simulink library "Lib_Piccolo"  (R2018b)
settings: Solver=VariableStepAuto  StartTime=0.0  StopTime=10.0  RelTol=1e-3
values from neighbouring files (symbols this model uses):
  AccelErrInt2Brakes = 0.15    [SimulationControlConfig16P.m]    (also in SimulationControlConfig16P_LEGACY.m; SimulationControlConfigTAILLESS.m = 0.2; SimulationControlConfigUTAIL.m = 0.2)
  AileronMax = 25    [SimulationControlConfig16P.m]    (also in SimulationControlConfig16P_LEGACY.m; SimulationControlConfigTAILLESS.m; SimulationControlConfigUTAIL.m)
  AileronPower = 0.00268    [SimulationControlConfig16P.m]    (also in SimulationControlConfig16P_LEGACY.m; SimulationControlConfigTAILLESS.m; SimulationControlConfigUTAIL.m)
  AileronSurfaceMax = 45    [SimulationControlConfig16P.m]    (also in SimulationControlConfig16P_LEGACY.m)
  AileronTrim = 0    [SimulationControlConfig16P.m]    (also in SimulationControlConfig16P_LEGACY.m; SimulationControlConfigTAILLESS.m; SimulationControlConfigUTAIL.m)
  Alt = 1000 + TerrainHeight    [SimulationStateConfig.m]
  AltCruise_m = testPlans(testIndx).terrainElevation * 0.3048 + 200    [SimulationControlConfig16P.m]    (also in SimulationControlConfigTAILLESS.m = 1083; SimulationControlConfigUTAIL.m = testPlans(testIndx).terrainElevation * 0.3048 + 152)
  AltitudeRate2PitchCmdIntegratorInit = 0.1    [SimulationControlPre.m]
  AltMax = 10000    [SimulationControlConfig16P.m]    (also in SimulationControlConfig16P_LEGACY.m; SimulationControlConfigTAILLESS.m; SimulationControlConfigUTAIL.m)
  AltMaxAccel = 1.25    [SimulationControlConfig16P.m]    (also in SimulationControlConfig16P_LEGACY.m = 0.9; SimulationControlConfigTAILLESS.m = 1.7; SimulationControlConfigUTAIL.m = 2)
  AltMin = 0    [SimulationControlConfig16P.m]    (also in SimulationControlConfig16P_LEGACY.m; SimulationControlConfigTAILLESS.m; SimulationControlConfigUTAIL.m)
  AltRateCmd2Pitch = 0.50    (= 0.5)    [SimulationControlConfig16P.m]    (also in SimulationControlConfig16P_LEGACY.m = 0.6; SimulationControlConfigTAILLESS.m = 0.2; SimulationControlConfigUTAIL.m = 0.3)
  AltRateError2Pitch = 0.40    (= 0.4)    [SimulationControlConfig16P.m]    (also in SimulationControlConfig16P_LEGACY.m; SimulationControlConfigTAILLESS.m = 0.55; SimulationControlConfigUTAIL.m = 0.55)
  AltRateErrorInt2Pitch = 0.50    (= 0.5)    [SimulationControlConfig16P.m]    (also in SimulationControlConfig16P_LEGACY.m = 0.45; SimulationControlConfigTAILLESS.m; SimulationControlConfigUTAIL.m = 0.75)
  AltRateLpfCutOff = 3    [SimulationControlConfig16P.m]    (also in SimulationControlConfig16P_LEGACY.m; SimulationControlConfigTAILLESS.m = 2; SimulationControlConfigUTAIL.m = 2)
  AutoNosegear2Rudder = 26    [SimulationControlConfig16P.m]    (also in SimulationControlConfig16P_LEGACY.m; SimulationControlConfigTAILLESS.m = 25.2; SimulationControlConfigUTAIL.m = 14)
  b = 5.54    [SimulationControlConfig16P.m]    (also in SimulationControlConfig16P_LEGACY.m; SimulationControlConfigTAILLESS.m = 2.37; SimulationControlConfigUTAIL.m = 2.37)
  Bank2AileronIntegratorInit = 0    [SimulationControlPre.m]
  BankMax_User = BankMax_User/180*pi    (= 0.523598775598)    [SimulationControlConfig16P.m]    (also in SimulationControlConfig16P_LEGACY.m; SimulationControlConfigTAILLESS.m = 0.610865238198; SimulationControlConfigUTAIL.m = 0.628318530718)
  baseLegFlaps = 20    [SimulationControlConfig16P.m]    (also in SimulationControlConfig16P_LEGACY.m = 0; SimulationControlConfigTAILLESS.m = 15; SimulationControlConfigUTAIL.m = 10)
  C = GeneticOpt.C    [SimulationCostFunction.m]
  c = Sw/b    (= 0.841696750903)    [SimulationControlConfig16P.m]    (also in SimulationControlConfig16P_LEGACY.m; SimulationControlConfigTAILLESS.m = 0.354008438819; SimulationControlConfigUTAIL.m = 0.354008438819)
  cell2WheelFactorMG = 5.98    [SimulationSensorConfig16P_LEGACY.m]
  cell2WheelFactorNG = 1    [SimulationSensorConfig16P_LEGACY.m]
  cellSatMaxMG = 15000    [SimulationSensorConfig16P.m]    (also in SimulationSensorConfig16P_LEGACY.m; SimulationSensorConfigTAILLESS7P.m; SimulationSensorConfigUTAIL7P.m)
  cellSatMaxNG = 1000    [SimulationSensorConfig16P.m]    (also in SimulationSensorConfig16P_LEGACY.m; SimulationSensorConfigTAILLESS7P.m; SimulationSensorConfigUTAIL7P.m)
  cellSatMinMG = -15000    [SimulationSensorConfig16P.m]    (also in SimulationSensorConfig16P_LEGACY.m; SimulationSensorConfigTAILLESS7P.m; SimulationSensorConfigUTAIL7P.m)
  cellSatMinNG = -1000    [SimulationSensorConfig16P.m]    (also in SimulationSensorConfig16P_LEGACY.m; SimulationSensorConfigTAILLESS7P.m; SimulationSensorConfigUTAIL7P.m)
  CL_Limit = CL_Max    (= 0.54)    [SimulationControlConfig16P.m]    (also in SimulationControlConfig16P_LEGACY.m; SimulationControlConfigTAILLESS.m; SimulationControlConfigUTAIL.m = 0.53)
  CL_Max = 0.54    [SimulationControlConfig16P.m]    (also in SimulationControlConfig16P_LEGACY.m; SimulationControlConfigTAILLESS.m; SimulationControlConfigUTAIL.m = 0.53)
  CL_Max_Nom = 0.465    [SimulationControlConfig16P.m]    (also in SimulationControlConfig16P_LEGACY.m; SimulationControlConfigTAILLESS.m = 0.39; SimulationControlConfigUTAIL.m)
  CL_Min = 0    [SimulationControlConfig16P.m]    (also in SimulationControlConfig16P_LEGACY.m; SimulationControlConfigTAILLESS.m; SimulationControlConfigUTAIL.m)
  ClimbMaxFraction = 0.35    [SimulationControlConfig16P.m]    (also in SimulationControlConfig16P_LEGACY.m = 0.24; SimulationControlConfigTAILLESS.m = 0.19; SimulationControlConfigUTAIL.m = 0.21)
  ClimboutMaxBank = 7.0    (= 7)    [SimulationControlConfig16P.m]    (also in SimulationControlConfig16P_LEGACY.m; SimulationControlConfigTAILLESS.m = 5; SimulationControlConfigUTAIL.m)
  ClimboutTimer = 7.0    (= 7)    [SimulationControlConfig16P.m]    (also in SimulationControlConfig16P_LEGACY.m; SimulationControlConfigTAILLESS.m; SimulationControlConfigUTAIL.m)
  dCl_per_dFlap = 0.005581818    [SimulationControlConfig16P.m]    (also in SimulationControlConfig16P_LEGACY.m = 0; SimulationControlConfigTAILLESS.m = 0; SimulationControlConfigUTAIL.m = 0)
  DecelerationCmd = 3.1    [SimulationControlConfig16P.m]    (also in SimulationControlConfig16P_LEGACY.m; SimulationControlConfigTAILLESS.m = 0.1; SimulationControlConfigUTAIL.m = 0.1)
  DeRotateLogicEndTimer = abs((NoseDownLimit_Deg-1)/DeRotateRamp_Dps)    [SimulationControlConfig16P.m]    (also in SimulationControlConfig16P_LEGACY.m; SimulationControlConfigTAILLESS.m; SimulationControlConfigUTAIL.m)
  DeRotateLogicHoldNoseUpTimer = 0.1    [SimulationControlConfig16P.m]    (also in SimulationControlConfig16P_LEGACY.m; SimulationControlConfigTAILLESS.m; SimulationControlConfigUTAIL.m)
  DeRotateLogicTimerTimeout = 2    [SimulationControlConfig16P.m]    (also in SimulationControlConfig16P_LEGACY.m; SimulationControlConfigTAILLESS.m; SimulationControlConfigUTAIL.m)
  DeRotateLowerCmdSaturation = 0    [SimulationControlConfig16P.m]    (also in SimulationControlConfig16P_LEGACY.m; SimulationControlConfigTAILLESS.m; SimulationControlConfigUTAIL.m)
  DeRotateRamp_Dps = 3    [SimulationControlConfig16P.m]    (also in SimulationControlConfig16P_LEGACY.m; SimulationControlConfigTAILLESS.m = 8; SimulationControlConfigUTAIL.m = 8)
  DeRotateUpperCmdSaturation = 7    [SimulationControlConfig16P.m]    (also in SimulationControlConfig16P_LEGACY.m; SimulationControlConfigTAILLESS.m; SimulationControlConfigUTAIL.m)
  DescentMaxFraction = 0.22    [SimulationControlConfig16P.m]    (also in SimulationControlConfig16P_LEGACY.m = 0.2; SimulationControlConfigTAILLESS.m = 0.17; SimulationControlConfigUTAIL.m = 0.17)
  DesktopSimTerrainOffset_m = 0.406    [SimulationAircraftConfig.m]
  downwindFlaps = 0    [SimulationControlConfig16P.m]    (also in SimulationControlConfig16P_LEGACY.m; SimulationControlConfigTAILLESS.m; SimulationControlConfigUTAIL.m)
  DP_init = 0.5*1.225*V_init^2    [SimulationControlConfig16P.m]    (also in SimulationControlConfig16P_LEGACY.m; SimulationControlConfigTAILLESS.m; SimulationControlConfigUTAIL.m)
  dscNoiseMG = 1    [SimulationSensorConfig16P_LEGACY.m]
  dscNoiseNG = 0.25    [SimulationSensorConfig16P_LEGACY.m]
  DSCnumBits = 24    [SimulationSensorConfig16P.m]    (also in SimulationSensorConfig16P_LEGACY.m; SimulationSensorConfigTAILLESS7P.m; SimulationSensorConfigUTAIL7P.m)
  DSCRangeMaxMG = 15000    [SimulationSensorConfig16P.m]    (also in SimulationSensorConfig16P_LEGACY.m; SimulationSensorConfigTAILLESS7P.m; SimulationSensorConfigUTAIL7P.m)
  DSCRangeMaxNG = 1000    [SimulationSensorConfig16P.m]    (also in SimulationSensorConfig16P_LEGACY.m; SimulationSensorConfigTAILLESS7P.m; SimulationSensorConfigUTAIL7P.m)
  DSCRangeMinMG = -15000    [SimulationSensorConfig16P.m]    (also in SimulationSensorConfig16P_LEGACY.m; SimulationSensorConfigTAILLESS7P.m; SimulationSensorConfigUTAIL7P.m)
  DSCRangeMinNG = -1000    [SimulationSensorConfig16P.m]    (also in SimulationSensorConfig16P_LEGACY.m; SimulationSensorConfigTAILLESS7P.m; SimulationSensorConfigUTAIL7P.m)
  dt = DLLSim.dt    [SimulationTimeStep.m]    (also in SimulationTrim.m = 0.02)
  EarlyTouchdownThreshold = 3.0    (= 3)    [SimulationControlConfig16P.m]    (also in SimulationControlConfig16P_LEGACY.m; SimulationControlConfigTAILLESS.m = 2.2; SimulationControlConfigUTAIL.m = 2.5)
  ElevatorDeflectionRate = 15    [SimulationControlConfig16P.m]    (also in SimulationControlConfig16P_LEGACY.m = 12; SimulationControlConfigTAILLESS.m = 10; SimulationControlConfigUTAIL.m = 12)
  ElevatorMax = 25    [SimulationControlConfig16P.m]    (also in SimulationControlConfig16P_LEGACY.m; SimulationControlConfigTAILLESS.m; SimulationControlConfigUTAIL.m)
  ElevatorPower = -0.002209    [SimulationControlConfig16P.m]    (also in SimulationControlConfig16P_LEGACY.m; SimulationControlConfigTAILLESS.m = -0.002956; SimulationControlConfigUTAIL.m = -0.00205983)
  ElevatorTrim = -3.5    [SimulationControlConfig16P.m]    (also in SimulationControlConfig16P_LEGACY.m; SimulationControlConfigTAILLESS.m = -6; SimulationControlConfigUTAIL.m = -8)
  elevonBias = 0    [SimulationControlConfig16P.m]    (also in SimulationControlConfig16P_LEGACY.m; SimulationControlConfigTAILLESS.m; SimulationControlConfigUTAIL.m)
  Enable_TAS_Protection = 0    [SimulationControlConfig16P.m]    (also in SimulationControlConfig16P_LEGACY.m; SimulationControlConfigTAILLESS.m; SimulationControlConfigUTAIL.m)
  EnableCrossTrackAbort = 1    [SimulationControlConfig16P.m]    (also in SimulationControlConfigTAILLESS.m; SimulationControlConfigUTAIL.m)
  EnergyBandwidth = 0.02    [SimulationControlConfig16P.m]    (also in SimulationControlConfig16P_LEGACY.m; SimulationControlConfigTAILLESS.m = 0.06; SimulationControlConfigUTAIL.m = 0.06)
  EngineLhFuelCut = 0    [SimulationAircraftConfig.m]
  EngineRhFuelCut = 0    [SimulationAircraftConfig.m]
  FastThrottleRate = 0.075    [SimulationControlConfig16P.m]    (also in SimulationControlConfig16P_LEGACY.m = 0.05; SimulationControlConfigTAILLESS.m = 0.1; SimulationControlConfigUTAIL.m = 0.1)
  FilterWarmUpTime = 2    [SimulationSensorConfig16P.m]    (also in SimulationSensorConfig16P_LEGACY.m; SimulationSensorConfigTAILLESS7P.m; SimulationSensorConfigUTAIL7P.m)
  finalApproachFlaps = 20    [SimulationControlConfig16P.m]    (also in SimulationControlConfig16P_LEGACY.m = 0; SimulationControlConfigTAILLESS.m = 22; SimulationControlConfigUTAIL.m = 10)
  FinalDescentSlope_Deg = testPlans(testIndx).descentSlope    [SimulationControlConfig16P.m]    (also in SimulationControlConfig16P_LEGACY.m; SimulationControlConfigTAILLESS.m; SimulationControlConfigUTAIL.m)
  flapMax = 0    [SimulationControlConfig16P.m]    (also in SimulationControlConfig16P_LEGACY.m; SimulationControlConfigTAILLESS.m; SimulationControlConfigUTAIL.m)
  flapRate = 7.5    [SimulationControlConfig16P.m]    (also in SimulationControlConfig16P_LEGACY.m; SimulationControlConfigTAILLESS.m = 6.6; SimulationControlConfigUTAIL.m)
  FlareHeight = 5    [SimulationControlConfig16P.m]    (also in SimulationControlConfig16P_LEGACY.m = 4.8; SimulationControlConfigTAILLESS.m = 2.5; SimulationControlConfigUTAIL.m = 2)
  FlareVerticalRate_mps = -0.4    [SimulationControlConfig16P.m]    (also in SimulationControlConfig16P_LEGACY.m = -0.5; SimulationControlConfigTAILLESS.m = -0.15; SimulationControlConfigUTAIL.m = -0.15)
  Fp_Aileron = 0.55*2*pi*RollRateLpfCutoff*dt    [SimulationControlConfig16P.m]    (also in SimulationControlConfig16P_LEGACY.m; SimulationControlConfigTAILLESS.m; SimulationControlConfigUTAIL.m)
  Fp_Alt = 0.55*AltBandwidth    (= 0.099)    [SimulationControlConfig16P.m]    (also in SimulationControlConfig16P_LEGACY.m; SimulationControlConfigTAILLESS.m = 0.587477826221; SimulationControlConfigUTAIL.m = 0.69115038379)
  Fp_AltRate = 0.55*2*pi*AltRateLpfCutOff*dt    [SimulationControlConfig16P.m]    (also in SimulationControlConfig16P_LEGACY.m; SimulationControlConfigTAILLESS.m; SimulationControlConfigUTAIL.m)
  Fp_Elevator = 0.55*2*pi*PitchRateLpfCutoff*dt    [SimulationControlConfig16P.m]    (also in SimulationControlConfig16P_LEGACY.m; SimulationControlConfigTAILLESS.m; SimulationControlConfigUTAIL.m)
  Fp_Energy = 0.55*2*pi*EnergyBandwidth    (= 0.069115038379)    [SimulationControlConfig16P.m]    (also in SimulationControlConfig16P_LEGACY.m; SimulationControlConfigTAILLESS.m = 0.207345115137; SimulationControlConfigUTAIL.m = 0.207345115137)
  Fp_Energy2 = 0.55*2*pi*EnergyBandwidth*dt    [SimulationControlConfig16P.m]    (also in SimulationControlConfig16P_LEGACY.m; SimulationControlConfigTAILLESS.m; SimulationControlConfigUTAIL.m)
  Fp_Pitch = 0.55*2*pi*PitchBandwidth    (= 2.76460153516)    [SimulationControlConfig16P.m]    (also in SimulationControlConfig16P_LEGACY.m = 3.11017672705; SimulationControlConfigTAILLESS.m = 3.80132711084; SimulationControlConfigUTAIL.m = 2.41902634326)
  Fp_Pitch_2 = 0.55*2*pi*PitchBandwidth*dt    [SimulationControlConfig16P.m]    (also in SimulationControlConfig16P_LEGACY.m; SimulationControlConfigTAILLESS.m; SimulationControlConfigUTAIL.m)
  Fp_Roll = RollBandwidth^2    (= 1)    [SimulationControlConfig16P.m]    (also in SimulationControlConfig16P_LEGACY.m = 1.44; SimulationControlConfigTAILLESS.m; SimulationControlConfigUTAIL.m)
  Fp_Rudder = 0.55*2*pi*YawRateLpfCutoff*dt    [SimulationControlConfig16P.m]    (also in SimulationControlConfig16P_LEGACY.m; SimulationControlConfigTAILLESS.m; SimulationControlConfigUTAIL.m)
  Fp_TAS = 0.55*2*pi*TASBandwidth    (= 0.103672557568)    [SimulationControlConfig16P.m]    (also in SimulationControlConfig16P_LEGACY.m; SimulationControlConfigTAILLESS.m = 0.172787595947; SimulationControlConfigUTAIL.m = 0.172787595947)
  Fp_TAS_Filter = 2*pi*TasLpfCutoff*dt    [SimulationControlConfig16P.m]    (also in SimulationControlConfig16P_LEGACY.m; SimulationControlConfigTAILLESS.m; SimulationControlConfigUTAIL.m)
  Fp_Turn = 0.55*2*pi*TurnErrLPFcutoff    (= 0.0345575191895)    [SimulationControlConfig16P.m]    (also in SimulationControlConfig16P_LEGACY.m; SimulationControlConfigTAILLESS.m = 0.172787595947; SimulationControlConfigUTAIL.m = 0.172787595947)
  Fp_TurnDerr = 0.55*2*pi*TurnDerivativeLPFcutoff    (= 0.0345575191895)    [SimulationControlConfig16P.m]    (also in SimulationControlConfig16P_LEGACY.m; SimulationControlConfigTAILLESS.m = 0.172787595947; SimulationControlConfigUTAIL.m = 0.172787595947)
  FTV = 3    [SimulationAircraftConfig.m]
  ftvStaticPositionError = 1/1.18    (= 0.847457627119)    [SimulationSensorConfig16P.m]    (also in SimulationSensorConfig16P_LEGACY.m; SimulationSensorConfigTAILLESS7P.m = 1; SimulationSensorConfigUTAIL7P.m = 1)
  g = 9.81    [SimulationStateConfig.m]
  GustSpd_Kts = testPlans(testIndx).gustSpd    [SimulationStateConfig.m]
  GustTriggerVal = testPlans(testIndx).gustTriggerVal    [SimulationStateConfig.m]
  HeadingErr2TurnRate = 0.5    [SimulationControlConfig16P.m]    (also in SimulationControlConfig16P_LEGACY.m; SimulationControlConfigTAILLESS.m; SimulationControlConfigUTAIL.m)
  HeadingErrDer2TurnRate = 0.3    [SimulationControlConfig16P.m]    (also in SimulationControlConfig16P_LEGACY.m; SimulationControlConfigTAILLESS.m; SimulationControlConfigUTAIL.m)
  IASbounce = IASstall*0.8    [SimulationControlPre.m]
  IAScruiseCMD = sqrt(2*m*9.81/(1.225*Sw*CL_cruise))    [SimulationControlConfig16P.m]    (also in SimulationControlConfig16P_LEGACY.m; SimulationControlConfigTAILLESS.m; SimulationControlConfigUTAIL.m)
  IASfinalCMD = 1.12 * IASmin    [SimulationControlConfig16P.m]    (also in SimulationControlConfig16P_LEGACY.m = 1.10 * IASmin; SimulationControlConfigTAILLESS.m = 1.10 * IASmin; SimulationControlConfigUTAIL.m = 1.15 * IASmin)
  IASflareCMD = IASstall    [SimulationControlConfig16P.m]    (also in SimulationControlConfig16P_LEGACY.m; SimulationControlConfigTAILLESS.m; SimulationControlConfigUTAIL.m)
  IASmax = 64    [SimulationControlConfig16P.m]    (also in SimulationControlConfig16P_LEGACY.m = 46; SimulationControlConfigTAILLESS.m = 38.58; SimulationControlConfigUTAIL.m = 35)
  IASmin = sqrt(2*m*9.81/(1.225*Sw*0.9*CL_Max_Nom))    [SimulationControlConfig16P.m]    (also in SimulationControlConfig16P_LEGACY.m; SimulationControlConfigTAILLESS.m; SimulationControlConfigUTAIL.m)
  IASshortCMD = IASstall    [SimulationControlConfig16P.m]    (also in SimulationControlConfig16P_LEGACY.m; SimulationControlConfigTAILLESS.m; SimulationControlConfigUTAIL.m)
  IASstall = sqrt(2*m*9.81/(1.225*Sw*CL_Max))    [SimulationControlConfig16P.m]    (also in SimulationControlConfig16P_LEGACY.m; SimulationControlConfigTAILLESS.m; SimulationControlConfigUTAIL.m)
  inFlight = 1    [SimulationControlConfig16P.m]    (also in SimulationControlConfigTAILLESS.m; SimulationControlConfigUTAIL.m)
  JetCatOffset = 5    [SimulationControlConfig16P.m]    (also in SimulationControlConfig16P_LEGACY.m)
  LaunchRollingElevator = -1.5    [SimulationControlConfig16P.m]    (also in SimulationControlConfig16P_LEGACY.m; SimulationControlConfigTAILLESS.m = 1; SimulationControlConfigUTAIL.m = 1)
  ldg_NosegearMax = 10    [SimulationControlConfig16P.m]    (also in SimulationControlConfig16P_LEGACY.m; SimulationControlConfigTAILLESS.m; SimulationControlConfigUTAIL.m)
  ldg_TrackVyErrInt2Nosegear = 0.1250    (= 0.125)    [SimulationControlConfig16P.m]    (also in SimulationControlConfig16P_LEGACY.m; SimulationControlConfigTAILLESS.m = 0.00714285714286; SimulationControlConfigUTAIL.m = 0.00714285714286)
  ldg_TrackVyErrPro2Nosegear = 0.35    [SimulationControlConfig16P.m]    (also in SimulationControlConfig16P_LEGACY.m; SimulationControlConfigTAILLESS.m = 0.0546666666667; SimulationControlConfigUTAIL.m = 0.0546666666667)
  ldg_TrackY2Vy = 0.07    [SimulationControlConfig16P.m]    (also in SimulationControlConfig16P_LEGACY.m; SimulationControlConfigTAILLESS.m = 0.17; SimulationControlConfigUTAIL.m = 0.17)
  ldg_Vy2NosegearScalingPower = 1.075    [SimulationControlConfig16P.m]    (also in SimulationControlConfig16P_LEGACY.m; SimulationControlConfigTAILLESS.m = 0.6; SimulationControlConfigUTAIL.m = 0.5)
  ldg_Y2VyScalingPower = 0.175    [SimulationControlConfig16P.m]    (also in SimulationControlConfig16P_LEGACY.m; SimulationControlConfigTAILLESS.m = 0; SimulationControlConfigUTAIL.m = 0)
  ldg_YawRate2Nosegear = 0.175    [SimulationControlConfig16P.m]    (also in SimulationControlConfig16P_LEGACY.m; SimulationControlConfigTAILLESS.m = 0.065; SimulationControlConfigUTAIL.m = 0.065)
  LiftSlope = 0.064285    [SimulationControlConfig16P.m]    (also in SimulationControlConfig16P_LEGACY.m; SimulationControlConfigTAILLESS.m = 0.058631; SimulationControlConfigUTAIL.m)
  LPFaileronInit = 0    [SimulationControlPre.m]
  LPFclestInit = 0    [SimulationControlPre.m]
  LPFenergyFFInit = 0    [SimulationControlPre.m]
  LPFtasInit = V_init + 2    [SimulationControlPre.m]
  LPFthrottleInit = ThrottleTrim    [SimulationControlPre.m]
  LPFturnErrInit = 0    [SimulationControlPre.m]
  ... (+115 more)
undefined symbols (not defined in the file or in its folder): abortFlag, alphaHPF, apmDelay, BRWNOUT, CRAWOR, CRAWUR, DiscIntNeverNeededParam, DLLSim, DLLSimStep, ECOMOR, ECOMUR, Fp_Tas, GustTrigger_HeightAgl_m, IPSTAT, LCINTEG, Ldg_Persist_Time, LOWER_FLAGS, MSG_ENABLE, NoiseStd, OLDVAL, OVERRIDE_ENABLE, OVERRIDE_VALUE, REBOOT, reversionEnable, revIASMax, revIASMin, revPitchMax, revPitchMin, revPitchRateMax, revRollMax, revRollRateMax, SAMPLE, SCALON, SensorModel, sigbuilder_block, Sim_Vx, Sim_Vy, Sim_Vz, Sim_Xpos, Sim_Ypos, Sim_Zpos, SYSOR, SYSUR, TARE, TEMPOR, TEMPUR, testIndx, testPlan, testPlans, Trim_piccoloInCmd, Trim_REFSI_FD_IN_nmodeCgShifterCmd_Ft, Trim_REFSI_FD_IN_nmodeFlapLhIBCmd_Deg, Trim_REFSI_FD_IN_nmodeFlapLhOBCmd_Deg, Trim_REFSI_FD_IN_nmodeFlapRhIBCmd_Deg, Trim_REFSI_FD_IN_nmodeFlapRhOBCmd_Deg, Trim_REFSI_FD_IN_nmodeSlatLhCmd_Deg, Trim_REFSI_FD_IN_nmodeSlatRhCmd_Deg, Trim_REFSI_FD_IN_nmodeSplrLhInbdCmd_Deg, Trim_REFSI_FD_IN_nmodeSplrLhOutbdCmd_Deg ... (+5)
libraries: simulink x866, aerolibconvert2 x60, $bdroot x52, aerolibatmos2 x5, dspswit3 x5, simulink_extras x4, dsparch4 x2, Lib_Piccolo_Alt x2, eeGeneralControl x1, dspindex x1
(part 3 of 44)

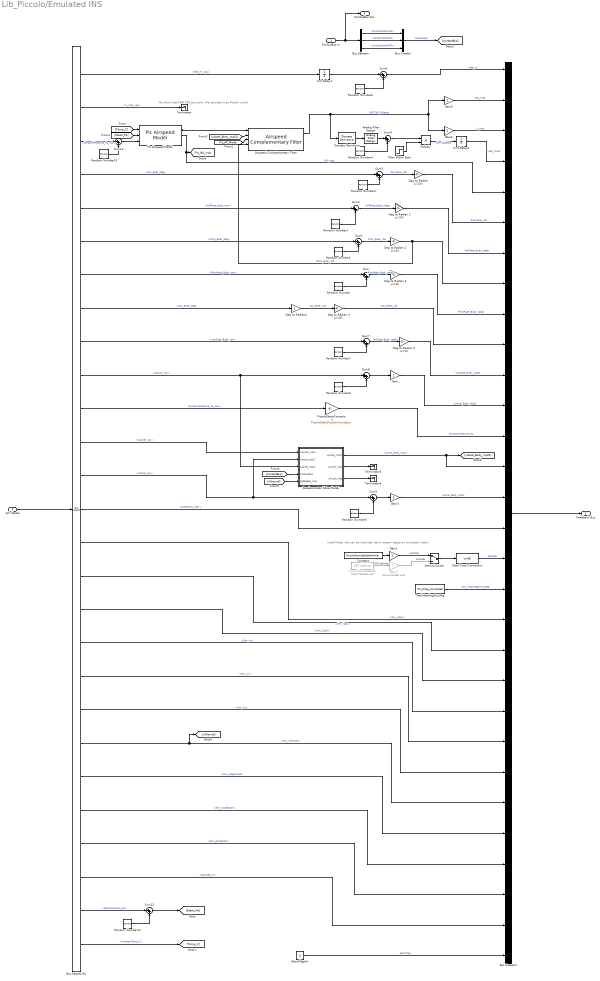
== system Lib_Piccolo/Emulated INS ==
  note: We Don't Use FDM TAS anymore. We calculate it as Piccolo would.
  note: Initial Mode, this can be overriden down stream based on simulation intent
  SimOutBus In : Inport
  A/C States : Inport  Port=2
  AbortFlagInit : Constant  Value=0
  Accelerometer Noise Model : Subsystem  VariantControl="sensorNoise == \"BASE\""
  Airspeed Complementary Filter : $bdroot/Airspeed Complementary Filter  SystemSampleTime=-1
  Analog Filter Design : dsparch4/Analog Filter Design  method=Butterworth  filttype=Lowpass  N=TASRateFilterOrder  Wlo=2*pi*TASRateCutOff  Whi=80  Rp=2  Rs=40
  Bus Creator : BusCreator  Inputs=3
  Bus Creator1 : BusCreator  Inputs=30
  Bus Selector : BusSelector  OutputSignals=GrndContactLMG,GrndContactNG,GrndContactRMG
  Bus Selector10 : BusSelector  OutputSignals=hdot_m_raw,V_mps_raw,DynamicPressure_Pa_raw,Roll_Euler_Deg,RollRate_Body_raw,Pitch_Euler_Deg,PitchRate_Body_raw,Yaw_Euler_Deg,YawRate_Body_raw,Zaccel_raw,DynamicPressure_Pa_raw,Xaccel_raw,Yaccel_raw,airDensity_kgm,Sim_Xpos,Sim_Ypos,Sim_Zpos,Sim_Vx,Sim_Vy,Sim_Vz,Sim_VGround,Sim_HdgGround,Sim_WindSouth,Sim_WindWest,altitude_m,StaticPressure_Pa,AmbientTemp_C
  Constant : Constant  Value=PiccoloStartingStateMachine  SampleTime=-1
  Data Type Conversion : DataTypeConversion  OutDataTypeStr=uint8
  Deg to Radian {,1..5} (6 alike) : Gain  Gain=pi/180
  Deg to Radian4 : Gain
  Discrete Derivative : simulink/Discrete/Discrete Derivative  gainval=1.0  ICPrevScaledInput=0.0  OutMin=[]  OutMax=[]  OutDataType=fixdt(1, 16)  OutScaling=2^-10  DoSatur=off
  Filter Warm Start : Step  Time=FilterWarmUpTime  SampleTime=0
  From Workspace25 : FromWorkspace  Commented=on  VariableName=REF.apMode  SampleTime=0
  Gain{,2..3,5} (4 alike) : Gain
  Gain1 : Gain  OutDataTypeStr=uint8
  Gain7 : Gain  Commented=on
  Manual Switch : ManualSwitch
  Multiply : Product
  Pic Airspeed Model : $bdroot/Pic Airspeed Model  correction=PiccoloStaticPositionCorrection
  PiccoloStaticCorrection : Gain  Gain=PiccoloStaticPositionCorrection
  Random Number : RandomNumber  Variance=NoiseStd.Q^2  SampleTime=dt
  Random Number1 : RandomNumber  Variance=NoiseStd.Pitch^2  SampleTime=dt
  Random Number12 : RandomNumber  Variance=NoiseStd.Static^2  SampleTime=dt
  Random Number13 : RandomNumber  Variance=NoiseStd.Dynamic^2  SampleTime=dt
  Random Number2 : RandomNumber  Variance=NoiseStd.P^2  SampleTime=dt
  Random Number3 : RandomNumber  Variance=NoiseStd.Roll^2  SampleTime=dt
  Random Number4 : RandomNumber  Variance=NoiseStd.TASRate^2  SampleTime=dt
  Random Number6 : RandomNumber  Variance=NoiseStd.VRate^2  SampleTime=dt
  Random Number7 : RandomNumber  Variance=NoiseStd.R^2  SampleTime=dt
  Random Number8 : RandomNumber  Variance=NoiseStd.ZAccel^2  SampleTime=dt
  Random Number9 : RandomNumber  Variance=NoiseStd.YAccel^2  SampleTime=dt
  Sum{,1..4,6..9,12..13} (11 alike) : Sum  Inputs=|++
  Terminator : Terminator
  Terminator3 : Terminator
  Terminator4 : Terminator
  TrackHeadingInit_Deg : Constant  Value=RwyHdg_Corrected
  Unit Delay1 : UnitDelay  SampleTime=-1
  Unit Delay3 : UnitDelay  SampleTime=-1
  SimOutBus Out : Outport
  Feedback Bus : Outport  Port=2
  tag scope: Pic_IAS_mps=global
  wires:
  Accelerometer Noise Model/3(zAccel_mps) -> Terminator4/1
  Accelerometer Noise Model/1(xAccel_mps2) -> Bus Creator1/14, [xAccel_Body_mps2]  "xAccel_Body_mps2"
  Accelerometer Noise Model/2(yAccel_mps) -> Terminator3/1
  [vGround] -> Accelerometer Noise Model/5(gndSpeed_mps)
  [contactBus] -> Accelerometer Noise Model/4(contactBus)
  Bus Creator/1 -> [contactBus]  "contactBus"
  Bus Selector/3 -> Bus Creator/3  "<GrndContactRMG>"
  Bus Selector/2 -> Bus Creator/2  "<GrndContactNG>"
  Bus Selector/1 -> Bus Creator/1  "<GrndContactLMG>"
  Bus Selector10/6 -> Sum1/1  "<Pitch_Euler_Deg>"
  Bus Selector10/7 -> Sum/1  "<PitchRate_Body_raw>"
  Bus Selector10/4 -> Sum3/1  "<Roll_Euler_Deg>"
  Sum6/1 -> Bus Creator1/1  "hdot_m"
  Unit Delay3/1 -> Bus Creator1/4  "Vdot_mps2"
  Deg to Radian 2/1 -> Airspeed Complementary Filter/4, Bus Creator1/8  "Pitch_Euler_rad"
  Deg to Radian 3/1 -> Bus Creator1/9  "PitchRate_Body_radps"
  Sum3/1 -> "Deg to Radian "/1  "Roll_Euler_rad"
  Gain/1 -> Bus Creator1/12  "zAccel_Body_mps2"
  Deg to Radian 1/1 -> Bus Creator1/7  "RollRate_Body_radps"
  Bus Selector10/5 -> Sum2/1  "<RollRate_Body_raw>"
  Bus Selector10/8 -> Deg to Radian4/1  "<Yaw_Euler_Deg>"
  Deg to Radian 5/1 -> Bus Creator1/11  "YawRate_Body_radps"
  Bus Selector10/9 -> Sum7/1  "<YawRate_Body_raw>"
  Deg to Radian 4/1 -> Bus Creator1/10  "Yaw_Euler_rad"
  Bus Creator1/1 -> Feedback Bus/1
  Bus Selector10/10 -> Sum8/1, Accelerometer Noise Model/3(Zaccel_mps2)  "<Zaccel_raw>"
  Bus Selector10/13 -> Accelerometer Noise Model/2(Yaccel_mps2), Sum9/1  "<Yaccel_raw>"
  Gain3/1 -> Bus Creator1/15  "yAccel_Body_mps2"
  A/C States/1 -> Bus Selector10/1
  Random Number1/1 -> Sum1/2
  Random Number2/1 -> Sum2/2
  Random Number3/1 -> Sum3/2
  Random Number4/1 -> Sum4/2
  Multiply/1 -> Unit Delay3/1  "Sim.TASRate"
  Random Number6/1 -> Sum6/2
  Random Number7/1 -> Sum7/2
  Random Number/1 -> Sum/2
  Discrete Derivative/1 -> Analog Filter Design/1
  "Deg to Radian "/1 -> Bus Creator1/6  "Roll_Euler_rad"
  Sum2/1 -> Deg to Radian 1/1  "RollRate_Body_radps"
  Sum1/1 -> Deg to Radian 2/1  "Pitch_Euler_rad"
  Sum/1 -> Deg to Radian 3/1  "PitchRate_Body_radps"
  Deg to Radian4/1 -> Deg to Radian 4/1  "Yaw_Euler_rad"
  Sum7/1 -> Deg to Radian 5/1  "YawRate_Body_radps"
  Sum8/1 -> Gain/1
  Random Number8/1 -> Sum8/2
  Sum9/1 -> Gain3/1
  Random Number9/1 -> Sum9/2
  Analog Filter Design/1 -> Sum4/1
  Filter Warm Start/1 -> Multiply/2
  Sum4/1 -> Multiply/1
  Bus Selector10/14 -> Bus Creator1/16  "<airDensity_kgm>"
  Bus Selector10/1 -> Unit Delay1/1  "<hdot_m_raw>"
  Bus Selector10/2 -> Terminator/1  "<V_mps_raw>"
  Airspeed Complementary Filter/1 -> Gain5/1, Gain2/1, Discrete Derivative/1  "REF.TAS_Filtered"
  Constant/1 -> Gain1/1
  Unit Delay1/1 -> Sum6/1
  Bus Selector10/12 -> Accelerometer Noise Model/1(XAccel_mps2)  "<Xaccel_raw>"
  Gain7/1 -> Manual Switch/2  "apMode"
  From Workspace25/1 -> Gain7/1  "REF.apMode"
  Gain1/1 -> Manual Switch/1  "apMode"
  Manual Switch/1 -> Data Type Conversion/1
  SimOutBus In/1 -> Bus Selector/1, SimOutBus Out/1
  Bus Selector10/15 -> Bus Creator1/19  "<Sim_Xpos>"
  Bus Selector10/16 -> Bus Creator1/20  "<Sim_Ypos>"
  Bus Selector10/17 -> Bus Creator1/21  "<Sim_Zpos>"
  Bus Selector10/18 -> Bus Creator1/22  "<Sim_Vx>"
  Bus Selector10/19 -> Bus Creator1/23  "<Sim_Vy>"
  Bus Selector10/20 -> Bus Creator1/24  "<Sim_Vz>"
  Bus Selector10/21 -> Bus Creator1/25, [vGround]  "<Sim_VGround>"
  Bus Selector10/22 -> Bus Creator1/26  "<Sim_HdgGround>"
  Bus Selector10/23 -> Bus Creator1/27  "<Sim_WindSouth>"
  Bus Selector10/24 -> Bus Creator1/28  "<Sim_WindWest>"
  Bus Selector10/25 -> Bus Creator1/29  "<altitude_m>"
  AbortFlagInit/1 -> Bus Creator1/30  "abortFlag"
  TrackHeadingInit_Deg/1 -> Bus Creator1/18  "Sim_TrackHdgCmd_Deg"
  Bus Selector10/26 -> Sum12/1  "<StaticPressure_Pa>"
  Bus Selector10/27 -> [Temp_C]  "<AmbientTemp_C>"
  [Temp_C] -> Pic Airspeed Model/1
  [Static_Pa] -> Pic Airspeed Model/2
  Bus Selector10/3 -> Sum13/1  "<DynamicPressure_Pa_raw>"
  PiccoloStaticCorrection/1 -> Bus Creator1/13  "DynamicPressure_Pa"
  Gain5/1 -> Bus Creator1/2  "TAS_mps"
  Bus Selector10/11 -> PiccoloStaticCorrection/1  "<DynamicPressure_Pa_raw>"
  Pic Airspeed Model/2 -> [Pic_IAS_mps], Bus Creator1/5  "IAS_mps"
  Pic Airspeed Model/1 -> Airspeed Complementary Filter/1
  [Pic_AP_Mode] -> Airspeed Complementary Filter/3
  [xAccel_Body_mps2] -> Airspeed Complementary Filter/2
  Sum12/1 -> [Static_Pa]
  Random Number12/1 -> Sum12/2
  Sum13/1 -> Pic Airspeed Model/3
  Random Number13/1 -> Sum13/2
  Gain2/1 -> Bus Creator1/3  "V_mps"
  Data Type Conversion/1 -> Bus Creator1/17  "apMode"

== system Lib_Piccolo/Emulated INS LEGACY ==
  note: Initial Mode, this can be overriden down stream based on simulation intent
  SimOutBus In : Inport
  A/C States : Inport  Port=2
  AbortFlagInit : Constant  Value=0
  Analog Filter Design : dsparch4/Analog Filter Design  method=Butterworth  filttype=Lowpass  N=TASRateFilterOrder  Wlo=2*pi*TASRateCutOff  Whi=80  Rp=2  Rs=40
  Bus Creator1 : BusCreator  Inputs=28
  Bus Selector10 : BusSelector  OutputSignals=hdot_m_raw,V_mps_raw,Roll_Euler_Deg,RollRate_Body_raw,Pitch_Euler_Deg,PitchRate_Body_raw,Yaw_Euler_Deg,YawRate_Body_raw,Zaccel_raw,DynamicPressure_Pa_raw,Xaccel_raw,Yaccel_raw,airDensity_kgm,Sim_Xpos,Sim_Ypos,Sim_Zpos,Sim_Vx,Sim_Vy,Sim_Vz,Sim_VGround,Sim_HdgGround,Sim_WindSouth,Sim_WindWest,altitude_m
  Constant : Constant  Value=PiccoloStartingStateMachine  SampleTime=-1
  Deg to Radian {,1..5} (6 alike) : Gain  Gain=pi/180
  Deg to Radian4 : Gain
  Discrete Derivative : simulink/Discrete/Discrete Derivative  gainval=1.0  ICPrevScaledInput=0.0  OutMin=[]  OutMax=[]  OutDataType=fixdt(1, 16)  OutScaling=2^-10  DoSatur=off
  Filter Warm Start : Step  Time=FilterWarmUpTime  SampleTime=0
  From Workspace25 : FromWorkspace  Commented=on  VariableName=REF.apMode  SampleTime=0
  Gain{,1..4} (5 alike) : Gain
  Gain7 : Gain  Commented=on
  LPF TAS : Subsystem
  Manual Switch : ManualSwitch
  Multiply : Product
  Random Number : RandomNumber  Variance=NoiseStd.Q^2  SampleTime=dt
  Random Number1 : RandomNumber  Variance=NoiseStd.Pitch^2  SampleTime=dt
  Random Number10 : RandomNumber  Variance=NoiseStd.XAccel^2  SampleTime=dt
  Random Number2 : RandomNumber  Variance=NoiseStd.P^2  SampleTime=dt
  Random Number3 : RandomNumber  Variance=NoiseStd.Roll^2  SampleTime=dt
  Random Number4 : RandomNumber  Variance=NoiseStd.TASRate^2  SampleTime=dt
  Random Number5 : RandomNumber  Variance=NoiseStd.TAS^2  SampleTime=dt
  Random Number6 : RandomNumber  Variance=NoiseStd.VRate^2  SampleTime=dt
  Random Number7 : RandomNumber  Variance=NoiseStd.R^2  SampleTime=dt
  Random Number8 : RandomNumber  Variance=NoiseStd.ZAccel^2  SampleTime=dt
  Random Number9 : RandomNumber  Variance=NoiseStd.YAccel^2  SampleTime=dt
  Sum{,1..10} (11 alike) : Sum  Inputs=|++
  TrackHeadingInit_Deg : Constant  Value=RwyHdg_Corrected
  Unit Delay1 : UnitDelay  SampleTime=-1
  Unit Delay3 : UnitDelay  SampleTime=-1
  SimOutBus Out : Outport
  Feedback Bus : Outport  Port=2
  tag scope: apMode=global
  wires:
  Bus Selector10/5 -> Sum1/1  "<Pitch_Euler_Deg>"
  Bus Selector10/6 -> Sum/1  "<PitchRate_Body_raw>"
  Bus Selector10/3 -> Sum3/1  "<Roll_Euler_Deg>"
  Bus Selector10/10 -> Gain2/1  "<DynamicPressure_Pa_raw>"
  Sum6/1 -> Bus Creator1/1  "hdot_m"
  Sum5/1 -> Bus Creator1/2  "V_mps"
  Unit Delay3/1 -> Bus Creator1/3  "Vdot_mps2"
  Deg to Radian 2/1 -> Bus Creator1/6  "Pitch_Euler_rad"
  Deg to Radian 3/1 -> Bus Creator1/7  "PitchRate_Body_radps"
  Sum3/1 -> "Deg to Radian "/1  "Roll_Euler_rad"
  Gain/1 -> Bus Creator1/10  "zAccel_Body_mps2"
  Gain2/1 -> Bus Creator1/11  "DynamicPressure_Pa"
  Deg to Radian 1/1 -> Bus Creator1/5  "RollRate_Body_radps"
  Bus Selector10/4 -> Sum2/1  "<RollRate_Body_raw>"
  Bus Selector10/7 -> Deg to Radian4/1  "<Yaw_Euler_Deg>"
  Deg to Radian 5/1 -> Bus Creator1/9  "YawRate_Body_radps"
  Bus Selector10/8 -> Sum7/1  "<YawRate_Body_raw>"
  Deg to Radian 4/1 -> Bus Creator1/8  "Yaw_Euler_rad"
  Bus Creator1/1 -> Feedback Bus/1
  Bus Selector10/9 -> Sum8/1  "<Zaccel_raw>"
  Bus Selector10/12 -> Sum9/1  "<Yaccel_raw>"
  Gain3/1 -> Bus Creator1/13  "yAccel_Body_mps2"
  A/C States/1 -> Bus Selector10/1
  Random Number1/1 -> Sum1/2
  Random Number2/1 -> Sum2/2
  Random Number3/1 -> Sum3/2
  Random Number4/1 -> Sum4/2
  Multiply/1 -> Unit Delay3/1  "Sim.TASRate"
  Random Number5/1 -> Sum5/2
  Random Number6/1 -> Sum6/2
  Random Number7/1 -> Sum7/2
  Random Number/1 -> Sum/2
  Discrete Derivative/1 -> Analog Filter Design/1
  "Deg to Radian "/1 -> Bus Creator1/4  "Roll_Euler_rad"
  Sum2/1 -> Deg to Radian 1/1  "RollRate_Body_radps"
  Sum1/1 -> Deg to Radian 2/1  "Pitch_Euler_rad"
  Sum/1 -> Deg to Radian 3/1  "PitchRate_Body_radps"
  Deg to Radian4/1 -> Deg to Radian 4/1  "Yaw_Euler_rad"
  Sum7/1 -> Deg to Radian 5/1  "YawRate_Body_radps"
  Sum8/1 -> Gain/1
  Random Number8/1 -> Sum8/2
  Sum9/1 -> Gain3/1
  Random Number9/1 -> Sum9/2
  Analog Filter Design/1 -> Sum4/1
  Filter Warm Start/1 -> Multiply/2
  Sum4/1 -> Multiply/1
  Bus Selector10/13 -> Bus Creator1/14  "<airDensity_kgm>"
  Bus Selector10/1 -> Unit Delay1/1  "<hdot_m_raw>"
  Bus Selector10/2 -> LPF TAS/1(Input)  "<V_mps_raw>"
  LPF TAS/1(Output) -> Discrete Derivative/1, Sum5/1  "REF.TAS_Filtered"
  Constant/1 -> Gain1/1
  Unit Delay1/1 -> Sum6/1
  Bus Selector10/11 -> Sum10/1  "<Xaccel_raw>"
  Random Number10/1 -> Sum10/2
  Sum10/1 -> Gain4/1
  Gain4/1 -> Bus Creator1/12  "xAccel_Body_mps2"
  Gain7/1 -> Manual Switch/2  "apMode"
  From Workspace25/1 -> Gain7/1  "REF.apMode"
  Gain1/1 -> Manual Switch/1  "apMode"
  Manual Switch/1 -> [apMode], Bus Creator1/15  "apMode"
  SimOutBus In/1 -> SimOutBus Out/1
  Bus Selector10/14 -> Bus Creator1/17  "<Sim_Xpos>"
  Bus Selector10/15 -> Bus Creator1/18  "<Sim_Ypos>"
  Bus Selector10/16 -> Bus Creator1/19  "<Sim_Zpos>"
  Bus Selector10/17 -> Bus Creator1/20  "<Sim_Vx>"
  Bus Selector10/18 -> Bus Creator1/21  "<Sim_Vy>"
  Bus Selector10/19 -> Bus Creator1/22  "<Sim_Vz>"
  Bus Selector10/20 -> Bus Creator1/23  "<Sim_VGround>"
  Bus Selector10/21 -> Bus Creator1/24  "<Sim_HdgGround>"
  Bus Selector10/22 -> Bus Creator1/25  "<Sim_WindSouth>"
  Bus Selector10/23 -> Bus Creator1/26  "<Sim_WindWest>"
  Bus Selector10/24 -> Bus Creator1/27  "<altitude_m>"
  AbortFlagInit/1 -> Bus Creator1/28  "abortFlag"
  TrackHeadingInit_Deg/1 -> Bus Creator1/16  "Sim_TrackHdgCmd_Deg"

== system Lib_Piccolo/Flap Deployment ==
  note: Switch on apMode to select flap setting
  FeedbackBus : Inport
  Bus Selector : BusSelector  OutputSignals=apMode
  Compare To Constant : simulink/Logic and Bit Operations/Compare To Constant  relop===  const=6  OutDataTypeStr=boolean
  Compare To Constant1 : simulink/Logic and Bit Operations/Compare To Constant  relop===  const=7  OutDataTypeStr=boolean
  Compare To Constant2 : simulink/Logic and Bit Operations/Compare To Constant  relop===  const=8  OutDataTypeStr=boolean
  Compare To Constant3 : simulink/Logic and Bit Operations/Compare To Constant  relop===  const=9  OutDataTypeStr=boolean
  Compare To Constant4 : simulink/Logic and Bit Operations/Compare To Constant  relop===  const=11  OutDataTypeStr=boolean
  Compare To Constant5 : simulink/Logic and Bit Operations/Compare To Constant  relop===  const=10  OutDataTypeStr=boolean
  Constant : Constant  Value=rolloutFlaps
  Constant1 : Constant  Value=shortFinalFlaps
  Constant2 : Constant  Value=finalApproachFlaps
  Constant3 : Constant  Value=baseLegFlaps
  Constant4 : Constant  Value=downwindFlaps
  Constant5 : Constant  Value=0
  OR : Logic  Operator=OR  IconShape=distinctive  AllPortsSameDT=off  OutDataTypeStr=boolean
  Rate Limiter : RateLimiter  RisingSlewLimit=flapRate  FallingSlewLimit=-flapRate  SampleTimeMode=inherited
  Saturation : Saturate  UpperLimit=flapMax  LowerLimit=0
  Switch{,1..4} (5 alike) : Switch  Criteria=u2 > Threshold  Threshold=0.5
  FlapCmd_deg : Outport
  tag scope: flapCmd=global
  wires:
  FeedbackBus/1 -> Bus Selector/1
  Bus Selector/1 -> Compare To Constant4/1, Compare To Constant5/1, Compare To Constant/1, Compare To Constant1/1, Compare To Constant2/1, Compare To Constant3/1  "<apMode>"
  Switch/1 -> Rate Limiter/1
  Compare To Constant/1 -> Switch4/2
  Compare To Constant4/1 -> Switch/2
  Constant/1 -> Switch/1
  OR/1 -> Switch1/2
  Switch1/1 -> Switch/3
  Constant1/1 -> Switch1/1
  Compare To Constant2/1 -> Switch2/2
  Switch2/1 -> Switch1/3
  Constant2/1 -> Switch2/1
  Compare To Constant1/1 -> Switch3/2
  Switch3/1 -> Switch2/3
  Constant3/1 -> Switch3/1
  Constant4/1 -> Switch4/1
  Switch4/1 -> Switch3/3
  Constant5/1 -> Switch4/3
  Saturation/1 -> [flapCmd], FlapCmd_deg/1
  Compare To Constant5/1 -> OR/1
  Compare To Constant3/1 -> OR/2
  Rate Limiter/1 -> Saturation/1

== system Lib_Piccolo/Ground Detection Systems ==
  SimOutputBus In : Inport
  " In 1" : Inport  Port=2
  CL Detection Wrapper : Subsystem
  Gain : Gain  Gain=2
  Gain1 : Gain  Gain=3
  OR : Logic  Operator=OR  IconShape=distinctive  AllPortsSameDT=off  OutDataTypeStr=boolean
  Terminator : Terminator
  Terminator1 : Terminator
  Unit Delay : UnitDelay  SampleTime=-1
  WoW Wrapper : Subsystem
  SimOutBus Out : Outport
  Feedback Bus : Outport  Port=2
  tag scope: TouchdownDetectedFlag=global
  wires:
  WoW Wrapper/2(WoWarmed) -> CL Detection Wrapper/1(WoWarmed)
  SimOutputBus In/1 -> SimOutBus Out/1, WoW Wrapper/1(SimBus)
  Gain1/1 -> Terminator1/1  "Sim_clContact"
  Gain/1 -> Terminator/1  "Sim_wowContact"
  OR/1 -> Unit Delay/1
  Unit Delay/1 -> [TouchdownDetectedFlag]  "Sim_TouchdownDetectedFlag"
  CL Detection Wrapper/1(TouchdownDetected) -> OR/2, Gain1/1
  WoW Wrapper/1(TouchdownDetected) -> Gain/1, OR/1
  " In 1"/1 -> Feedback Bus/1, CL Detection Wrapper/2(FeedbackBus), WoW Wrapper/2(FeedbackBus)

== system Lib_Piccolo/Guidance FLIGHT LEGACY ==
  SimOutBus In : Inport
  In1 : Inport  Port=2
  Bus Assignment : BusAssignment  AssignedSignals=Sim_Ypos,Sim_Vy,Sim_Zpos,Sim_Vz,Sim_Xpos,Sim_Vx,abortFlag
  Bus Selector : BusSelector  OutputSignals=VEarthFtps_0,VEarthFtps_1,VEarthFtps_2,XposnFt,YposnFt,ZposnFt
  Bus Selector1 : BusSelector  OutputSignals=abortFlag,Sim_TrackHdgCmd_Deg
  Ft to m{,1..5} (6 alike) : Gain  Gain=0.3048
  Track Position Decomposition : Subsystem
  Unit Delay{1..6} (6 alike) : UnitDelay  SampleTime=-1
  SimOutBus Out : Outport
  Out1 : Outport  Port=2
  wires:
  In1/1 -> Bus Selector1/1, Bus Assignment/1
  Bus Assignment/1 -> Out1/1
  Track Position Decomposition/2("Sim.Vy ") -> Bus Assignment/3  "Sim_Vy"
  SimOutBus In/1 -> Bus Selector/1, SimOutBus Out/1
  Bus Selector/1 -> Unit Delay5/1  "<VEarthFtps_0>"
  Bus Selector/2 -> Unit Delay1/1  "<VEarthFtps_1>"
  Bus Selector/4 -> Unit Delay2/1  "<XposnFt>"
  Bus Selector/5 -> Unit Delay3/1  "<YposnFt>"
  Ft to m/1 -> Track Position Decomposition/3(VNorth_mps)
  Ft to m1/1 -> Track Position Decomposition/4(VEast_mps)
  Ft to m2/1 -> Track Position Decomposition/6("Xposn_m ")  "Xposn_m"
  Ft to m3/1 -> Track Position Decomposition/7(Yposn_m)  "Yposn_m"
  Track Position Decomposition/1(Sim.Ypos) -> Bus Assignment/2  "Sim_Ypos"
  Unit Delay5/1 -> Ft to m/1
  Unit Delay1/1 -> Ft to m1/1
  Unit Delay2/1 -> Ft to m2/1
  Unit Delay3/1 -> Ft to m3/1
  Bus Selector/3 -> Unit Delay4/1  "<VEarthFtps_2>"
  Unit Delay4/1 -> Ft to m4/1
  Ft to m4/1 -> Track Position Decomposition/5(VDown_mps)
  Bus Selector/6 -> Unit Delay6/1  "<ZposnFt>"
  Unit Delay6/1 -> Ft to m5/1
  Ft to m5/1 -> Track Position Decomposition/8(Zposn_m)  "Zposn_m"
  Track Position Decomposition/3(Sim.Zpos) -> Bus Assignment/4  "Sim_Zpos"
  Track Position Decomposition/4(Sim.Vz) -> Bus Assignment/5  "Sim_Vz"
  Track Position Decomposition/5(Sim.Xpos) -> Bus Assignment/6  "Sim_Xpos"
  Track Position Decomposition/6(Sim.Vx) -> Bus Assignment/7  "Sim_Vx"
  Bus Selector1/1 -> Track Position Decomposition/1(abortFlag)  "<abortFlag>"
  Track Position Decomposition/7(Sim.abortFlag) -> Bus Assignment/8  "Sim_abortFlag"
  Bus Selector1/2 -> Track Position Decomposition/2(TrackHeading_Deg)  "<Sim_TrackHdgCmd_Deg>"

== system Lib_Piccolo/Guidance LDG ==
  SimOutBus In : Inport
  In1 : Inport  Port=2
  Bus Assignment : BusAssignment  AssignedSignals=Sim_Ypos,Sim_Vy,Sim_Zpos,Sim_Vz,Sim_Xpos,Sim_Vx,abortFlag
  Bus Selector : BusSelector  OutputSignals=VEarthFtps_0,VEarthFtps_1,VEarthFtps_2,XposnFt,YposnFt,ZposnFt
  Bus Selector1 : BusSelector  OutputSignals=apMode,Sim_VGround,abortFlag,Sim_TrackHdgCmd_Deg
  Ft to m{,1..5} (6 alike) : Gain  Gain=0.3048
  Track Position Decomposition : Subsystem
  Unit Delay{1..6} (6 alike) : UnitDelay  SampleTime=-1
  SimOutBus Out : Outport
  Out1 : Outport  Port=2
  wires:
  In1/1 -> Bus Selector1/1, Bus Assignment/1
  Bus Assignment/1 -> Out1/1
  Track Position Decomposition/2("Sim.Vy ") -> Bus Assignment/3  "Sim_Vy"
  SimOutBus In/1 -> Bus Selector/1, SimOutBus Out/1
  Bus Selector/1 -> Unit Delay5/1  "<VEarthFtps_0>"
  Bus Selector/2 -> Unit Delay1/1  "<VEarthFtps_1>"
  Bus Selector/4 -> Unit Delay2/1  "<XposnFt>"
  Bus Selector/5 -> Unit Delay3/1  "<YposnFt>"
  Ft to m/1 -> Track Position Decomposition/5(VNorth_mps)
  Ft to m1/1 -> Track Position Decomposition/6(VEast_mps)
  Ft to m2/1 -> Track Position Decomposition/8("Xposn_m ")  "Xposn_m"
  Ft to m3/1 -> Track Position Decomposition/9(Yposn_m)  "Yposn_m"
  Track Position Decomposition/1(Sim.Ypos) -> Bus Assignment/2  "Sim_Ypos"
  Unit Delay5/1 -> Ft to m/1
  Unit Delay1/1 -> Ft to m1/1
  Unit Delay2/1 -> Ft to m2/1
  Unit Delay3/1 -> Ft to m3/1
  Bus Selector/3 -> Unit Delay4/1  "<VEarthFtps_2>"
  Unit Delay4/1 -> Ft to m4/1
  Ft to m4/1 -> Track Position Decomposition/7(VDown_mps)
  Bus Selector/6 -> Unit Delay6/1  "<ZposnFt>"
  Unit Delay6/1 -> Ft to m5/1
  Ft to m5/1 -> Track Position Decomposition/10(Zposn_m)  "Zposn_m"
  Track Position Decomposition/3(Sim.Zpos) -> Bus Assignment/4  "Sim_Zpos"
  Track Position Decomposition/4(Sim.Vz) -> Bus Assignment/5  "Sim_Vz"
  Track Position Decomposition/5(Sim.Xpos) -> Bus Assignment/6  "Sim_Xpos"
  Track Position Decomposition/6(Sim.Vx) -> Bus Assignment/7  "Sim_Vx"
  Bus Selector1/1 -> Track Position Decomposition/1(apMode)  "<apMode>"
  Bus Selector1/2 -> Track Position Decomposition/2(VGround_mps)  "<Sim_VGround>"
  Bus Selector1/3 -> Track Position Decomposition/3(abortFlag)  "<abortFlag>"
  Track Position Decomposition/7(Sim.abortFlag) -> Bus Assignment/8  "Sim_abortFlag"
  Bus Selector1/4 -> Track Position Decomposition/4(TrackHeading_Deg)  "<Sim_TrackHdgCmd_Deg>"

== system Lib_Piccolo/Guidance Takeoff & Flight ==
  SimOutBus In : Inport
  In1 : Inport  Port=2
  Bus Assignment : BusAssignment  AssignedSignals=Sim_Ypos,Sim_Vy,Sim_Zpos,Sim_Vz,Sim_Xpos,Sim_Vx,abortFlag
  Bus Selector : BusSelector  OutputSignals=VEarthFtps_0,VEarthFtps_1,VEarthFtps_2,XposnFt,YposnFt,ZposnFt
  Bus Selector1 : BusSelector  OutputSignals=apMode,Sim_VGround,abortFlag,Sim_TrackHdgCmd_Deg
  Ft to m{,1..5} (6 alike) : Gain  Gain=0.3048
  Track Position Decomposition : Subsystem
  Unit Delay{1..6} (6 alike) : UnitDelay  SampleTime=-1
  SimOutBus Out : Outport
  Out1 : Outport  Port=2
  wires:
  In1/1 -> Bus Selector1/1, Bus Assignment/1
  Bus Assignment/1 -> Out1/1
  Track Position Decomposition/2("Sim.Vy ") -> Bus Assignment/3  "Sim_Vy"
  SimOutBus In/1 -> Bus Selector/1, SimOutBus Out/1
  Bus Selector/1 -> Unit Delay5/1  "<VEarthFtps_0>"
  Bus Selector/2 -> Unit Delay1/1  "<VEarthFtps_1>"
  Bus Selector/4 -> Unit Delay2/1  "<XposnFt>"
  Bus Selector/5 -> Unit Delay3/1  "<YposnFt>"
  Ft to m/1 -> Track Position Decomposition/5(VNorth_mps)
  Ft to m1/1 -> Track Position Decomposition/6(VEast_mps)
  Ft to m2/1 -> Track Position Decomposition/8("Xposn_m ")  "Xposn_m"
  Ft to m3/1 -> Track Position Decomposition/9(Yposn_m)  "Yposn_m"
  Track Position Decomposition/1(Sim.Ypos) -> Bus Assignment/2  "Sim_Ypos"
  Unit Delay5/1 -> Ft to m/1
  Unit Delay1/1 -> Ft to m1/1
  Unit Delay2/1 -> Ft to m2/1
  Unit Delay3/1 -> Ft to m3/1
  Bus Selector/3 -> Unit Delay4/1  "<VEarthFtps_2>"
  Unit Delay4/1 -> Ft to m4/1
  Ft to m4/1 -> Track Position Decomposition/7(VDown_mps)
  Bus Selector/6 -> Unit Delay6/1  "<ZposnFt>"
  Unit Delay6/1 -> Ft to m5/1
  Ft to m5/1 -> Track Position Decomposition/10(Zposn_m)  "Zposn_m"
  Track Position Decomposition/3(Sim.Zpos) -> Bus Assignment/4  "Sim_Zpos"
  Track Position Decomposition/4(Sim.Vz) -> Bus Assignment/5  "Sim_Vz"
  Track Position Decomposition/5(Sim.Xpos) -> Bus Assignment/6  "Sim_Xpos"
  Track Position Decomposition/6(Sim.Vx) -> Bus Assignment/7  "Sim_Vx"
  Bus Selector1/1 -> Track Position Decomposition/1(apMode)  "<apMode>"
  Bus Selector1/2 -> Track Position Decomposition/2(VGround_mps)  "<Sim_VGround>"
  Bus Selector1/3 -> Track Position Decomposition/3(abortFlag)  "<abortFlag>"
  Track Position Decomposition/7(Sim.abortFlag) -> Bus Assignment/8  "Sim_abortFlag"
  Bus Selector1/4 -> Track Position Decomposition/4(TrackHeading_Deg)  "<Sim_TrackHdgCmd_Deg>"

== system Lib_Piccolo/Heading Control ==
  note: Not sure how this works :S. Where is wind compensation added?
  note: Two versions of control here. There is a track following control and heading following control.
  Heading : Inport
  TrackY : Inport  Port=2
  Feedback Bus : Inport  Port=3
  BankCmd_Euler_Deg : Constant  Commented=on  Value=0
  Bus Selector1 : BusSelector  OutputSignals=Sim_HdgGround,Sim_VGround,V_mps,apMode,Roll_Euler_rad
  Bus Selector2 : BusSelector  OutputSignals=Yaw_Euler_rad,Sim_HdgGround,Sim_VGround,Sim_WindSouth,Sim_WindWest,Sim_TrackHdgCmd_Deg
  Constant2 : Constant  Value=0
  Convergence : Gain  Gain=TrackConvergence/100
  Deg2Rad : Gain  Gain=pi/180
  Deg2Rad1 : Gain  Commented=on  Gain=pi/180
  Derivative : Derivative
  Divide6 : Product  Inputs=**/
  From Workspace24 : FromWorkspace  Commented=on  VariableName=REF.WindSouth  SampleTime=0
  From Workspace29 : FromWorkspace  Commented=on  VariableName=REF.WindWest  SampleTime=0
  Gain1 : Gain  Gain=89/90
  Kd_Turn : Gain  Gain=HeadingErrDer2TurnRate
  Kp_Turn : Gain  Gain=HeadingErr2TurnRate
  LPF Heading : Subsystem
  LPF HeadingDerivative : Subsystem
  Manual Switch1 : ManualSwitch
  On Ground : Subsystem
  Rad2Deg : Gain  Gain=180/pi
  Rad2Deg1 : Gain  Commented=on  Gain=180/pi
  Rad2Deg2 : Gain  Gain=180/pi
  Saturation : Saturate  UpperLimit=90  LowerLimit=-90
  Sum : Sum  Inputs=|+-
  Sum1 : Sum  Inputs=|++
  Sum2 : Sum  Inputs=+-|
  Sum4 : Sum  Commented=on  Inputs=+-|
  Switch : Switch  Criteria=u2 > Threshold  Threshold=0.5
  Terminator : Terminator
  Terminator1 : Terminator
  Terminator2 : Terminator
  Trigonometric Function1 : Trigonometry  Operator=atan
  Trigonometric Function2 : Trigonometry  Operator=atan
  UnwindHdg : Subsystem  Commented=on
  UnwindHdg1 : Subsystem  Commented=on
  WindCorrectionEstimate : Subsystem  Commented=on
  g2 : Constant  Value=9.81
  BankCmd : Outport
  SideSlipCmd : Outport  Port=2
  tag scope: Sim_SideSlipCmd=global
  wires:
  Feedback Bus/1 -> Bus Selector1/1, Bus Selector2/1
  TrackY/1 -> Convergence/1
  Deg2Rad/1 -> Divide6/1
  Bus Selector1/2 -> Divide6/2  "<Sim_VGround>"
  g2/1 -> Divide6/3
  Divide6/1 -> Trigonometric Function2/1
  Heading/1 -> Manual Switch1/2  "HeadingOnly_Deg"
  Bus Selector1/1 -> Sum/2  "<Sim_HdgGround>"
  Derivative/1 -> LPF HeadingDerivative/1(Input)
  Kp_Turn/1 -> Sum1/1
  Sum1/1 -> Deg2Rad/1
  Convergence/1 -> Trigonometric Function1/1  "Convergence"
  LPF HeadingDerivative/1(Output) -> Kd_Turn/1  "TurnErrDerivativeFilter"
  Trigonometric Function2/1 -> LPF Heading/1(Input)
  Kd_Turn/1 -> Sum1/2
  Sum2/1 -> Manual Switch1/1  "Sim.TrackerHdgCmd"
  Sum/1 -> Derivative/1, Kp_Turn/1  "Sim.Hdg Error"
  Gain1/1 -> Saturation/1
  From Workspace24/1 -> ?  "REF.WindSouth"
  From Workspace29/1 -> ?  "REF.WindWest"
  Rad2Deg/1 -> Gain1/1
  Manual Switch1/1 -> Sum/1
  Trigonometric Function1/1 -> Rad2Deg/1
  Saturation/1 -> Sum2/2  "TrackerHdgDeltaCmd"
  Bus Selector2/6 -> Sum2/1  "<Sim_TrackHdgCmd_Deg>"
  Bus Selector2/4 -> WindCorrectionEstimate/1(WindSouth)  "<Sim_WindSouth>"
  Bus Selector2/5 -> WindCorrectionEstimate/2(WindWest)  "<Sim_WindWest>"
  Bus Selector2/1 -> Rad2Deg1/1  "<Yaw_Euler_rad>"
  Bus Selector2/2 -> Sum4/2  "<Sim_HdgGround>"
  Rad2Deg1/1 -> Sum4/1
  Constant2/1 -> SideSlipCmd/1, [Sim_SideSlipCmd]  "Sim_SideSlipCmd"
  BankCmd_Euler_Deg/1 -> Deg2Rad1/1  "Sim.RollCmd"
  Rad2Deg2/1 -> Terminator/1  "Sim.BankCmd"
  Switch/1 -> Rad2Deg2/1, BankCmd/1  "Sim_BankCmd"
  Bus Selector2/3 -> Terminator1/1  "<Sim_VGround>"
  LPF Heading/1(Output) -> On Ground/1(GuidanceBankCmd)  "Sim_BankCmd"
  Bus Selector1/4 -> On Ground/2(<apMode>)  "<apMode>"
  Bus Selector1/3 -> Terminator2/1  "<V_mps>"
  On Ground/1(BankCmd) -> Switch/1
  [ApGlobal] -> Switch/2
  Bus Selector1/5 -> Switch/3  "<Roll_Euler_rad>"
